simulink subsystem "Admittance_Controller_6D"  (R2025b)
settings: Solver=VariableStepAuto  StartTime=0.0  StopTime=10.0  RelTol=1e-3
values from neighbouring files (symbols this model uses):
  A6 = (2*M - D*Ts) ./ (2*M + D*Ts)    [setup_handguiding_lab.m]
  B6 = Ts ./ (2*M + D*Ts)    [setup_handguiding_lab.m]
settings Model: Creator=Compu  LastModifiedBy=Compu

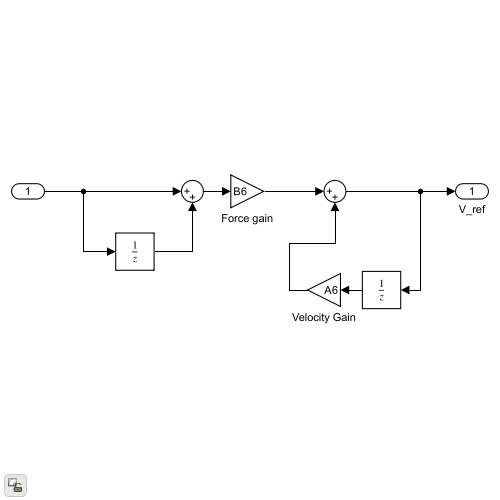
[thumbnail: Simulink's stored preview of the top-level diagram]
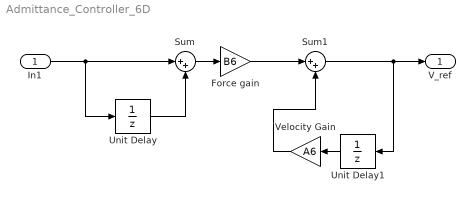
== system Admittance_Controller_6D ==
  In1 : Inport
  Force gain : Gain  Gain=B6
  Sum : Sum  Inputs=|++
  Sum1 : Sum  Inputs=|++
  Unit Delay : UnitDelay  InitialCondition=zeros(6,1)  SampleTime=0.002  HasFrameUpgradeWarning=on
  Unit Delay1 : UnitDelay  InitialCondition=zeros(6,1)  SampleTime=0.002  HasFrameUpgradeWarning=on
  Velocity Gain : Gain  Gain=A6
  V_ref : Outport
  wires:
  Sum/1 -> Force gain/1
  Sum1/1 -> Unit Delay1/1, V_ref/1
  Unit Delay1/1 -> Velocity Gain/1
  Velocity Gain/1 -> Sum1/2
  In1/1 -> Unit Delay/1, Sum/1
  Unit Delay/1 -> Sum/2
  Force gain/1 -> Sum1/1
